simulink model "clik_second_order"  (R2023a)
settings: Solver=VariableStepAuto  StartTime=0.0  StopTime=24*5  RelTol=1e-3
undefined symbols (not defined in the file or in its folder): DiscIntNeverNeededParam, Kd, Kp, q0, Tc
settings Model: Creator=Valentina Giannotti  LastModifiedBy=salpi
settings OptimizationCC: ReuseModelBlockBuffer=off

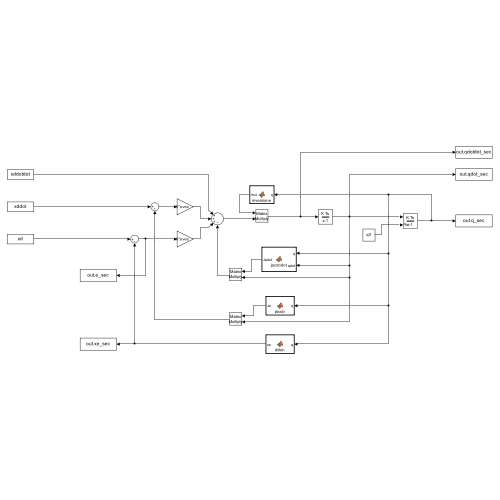
[thumbnail: Simulink's stored preview of the top-level diagram]
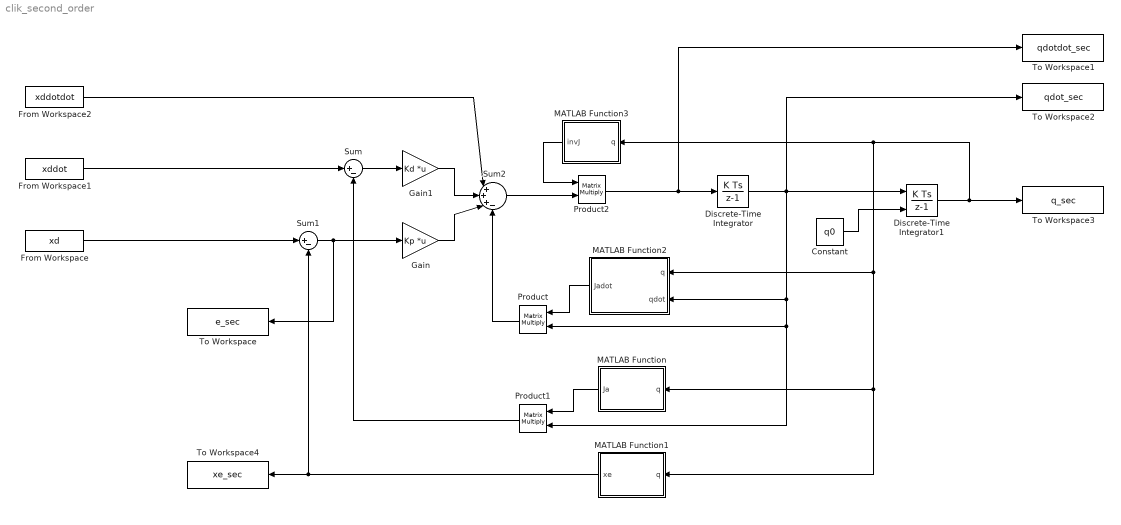
== system clik_second_order ==
  Constant : Constant  Value=q0
  Discrete-Time Integrator : DiscreteIntegrator  InitialCondition=[0 0 0 0]'  SampleTime=Tc  ICPrevOutput=DiscIntNeverNeededParam  ICPrevScaledInput=DiscIntNeverNeededParam
  Discrete-Time Integrator1 : DiscreteIntegrator  InitialConditionSource=external  SampleTime=Tc  ICPrevOutput=DiscIntNeverNeededParam  ICPrevScaledInput=DiscIntNeverNeededParam
  From Workspace : FromWorkspace  VariableName=xd
  From Workspace1 : FromWorkspace  VariableName=xddot
  From Workspace2 : FromWorkspace  VariableName=xddotdot
  Gain : Gain  Gain=Kp  Multiplication=Matrix(K*u) (u vector)
  Gain1 : Gain  Gain=Kd  Multiplication=Matrix(K*u) (u vector)
  MATLAB Function : MATLAB Function  TreatAsAtomicUnit=on
  MATLAB Function1 : MATLAB Function  TreatAsAtomicUnit=on
  MATLAB Function2 : MATLAB Function  TreatAsAtomicUnit=on
  MATLAB Function3 : MATLAB Function  TreatAsAtomicUnit=on
  Product : Product  Multiplication=Matrix(*)
  Product1 : Product  Multiplication=Matrix(*)
  Product2 : Product  Multiplication=Matrix(*)
  Sum : Sum  Inputs=|+-
  Sum1 : Sum  Inputs=|+-
  Sum2 : Sum  Inputs=|+++-
  To Workspace : ToWorkspace  VariableName=e_sec  SaveFormat=Structure With Time  SampleTime=-1
  To Workspace1 : ToWorkspace  VariableName=qdotdot_sec  SaveFormat=Structure With Time  SampleTime=-1
  To Workspace2 : ToWorkspace  VariableName=qdot_sec  SaveFormat=Structure With Time  SampleTime=-1
  To Workspace3 : ToWorkspace  VariableName=q_sec  SaveFormat=Structure With Time  SampleTime=-1
  To Workspace4 : ToWorkspace  VariableName=xe_sec  SaveFormat=Structure With Time  SampleTime=-1
  wires:
  Sum2/1 -> Product2/2
  From Workspace/1 -> Sum1/1
  Constant/1 -> Discrete-Time Integrator1/2
  Discrete-Time Integrator/1 -> To Workspace2/1, Discrete-Time Integrator1/1, Product1/2, Product/2, MATLAB Function2/2(qdot)
  From Workspace1/1 -> Sum/1
  Product/1 -> Sum2/4
  Sum1/1 -> Gain/1, To Workspace/1
  MATLAB Function3/1(invJ) -> Product2/1
  MATLAB Function1/1(xe) -> To Workspace4/1, Sum1/2
  Gain1/1 -> Sum2/2
  MATLAB Function2/1(Jadot) -> Product/1
  Discrete-Time Integrator1/1 -> MATLAB Function3/1(q), MATLAB Function/1(q), MATLAB Function1/1(q), MATLAB Function2/1(q), To Workspace3/1
  MATLAB Function/1(Ja) -> Product1/1
  Gain/1 -> Sum2/3
  From Workspace2/1 -> Sum2/1
  Product2/1 -> Discrete-Time Integrator/1, To Workspace1/1
  Sum/1 -> Gain1/1
  Product1/1 -> Sum/2

== matlab function clik_second_order/MATLAB Function ==
  data: q input; Ja output
function Ja = jacob(q)
% Map joint rates to [x_dot; y_dot; z_dot; phi_dot].

a1=0.5;
a2=a1;
d0=1;

Ja = [-a1*sin(q(1))-a2*sin(q(1)+q(2)),-a2*sin(q(1)+q(2)),0,0;
       a1*cos(q(1))+a2*cos(q(1)+q(2)),a2*cos(q(1)+q(2)),0,0;
       0,0,1,0;
       1,1,0,1];

end

== matlab function clik_second_order/MATLAB Function2 ==
  data: q input; Jadot output; qdot input
function Jadot = jacobdot(q,qdot)
% Only the planar rows change with the joint angles.

a1=0.5;
a2=a1;

Jadot = [qdot(1)*(-a1*cos(q(1)))-(qdot(1)+qdot(2))*a2*cos(q(1)+q(2)),(qdot(1)+qdot(2))*(-a2*cos(q(1)+q(2))),0,0;
         qdot(1)*(-a1*sin(q(1)))-(qdot(1)+qdot(2))*a2*sin(q(1)+q(2)),(qdot(1)+qdot(2))*(-a2*sin(q(1)+q(2))),0,0;
         0,0,0,0;
         0,0,0,0];
end

== matlab function clik_second_order/MATLAB Function3 ==
  data: invJ output; q input
function invJ=inversione(q)
% Map the full pose correction back to joint space.
a1=0.5;
a2=a1;

J=[-a1*sin(q(1))-a2*sin(q(1)+q(2)),-a2*sin(q(1)+q(2)),0,0;...
    a1*cos(q(1))+a2*cos(q(1)+q(2)),a2*cos(q(1)+q(2)),0,0;...
    0,0,1,0;...
    1,1,0,1];
invJ=J^-1;
end

== matlab function clik_second_order/MATLAB Function1 ==
  data: q input; xe output
function xe = dirkin(q)
% Pose in base coordinates, ordered as [x; y; z; phi].
a1=0.5;
a2=a1;
d0=1;

xe=[a1*cos(q(1))+a2*cos(q(1)+q(2));...
    a1*sin(q(1))+a2*sin(q(1)+q(2));...
    d0+q(3);...
    q(1)+q(2)+q(4)];
end
